simulink model "HybridControllerP2C2ahm"  (R2024b)
settings: Solver=FixedStepDiscrete  StartTime=0.0  StopTime=inf  FixedStep=controlPeriod  RelTol=1e-3
PreLoadFcn:
  | initializeSimulation;
InitFcn:
  | clear('all');
  | initializeSimulation;
values from neighbouring files (symbols this model uses):
  MRC = [2 0.05 0.001]./10    [ATS_setup.m]
  Nl = floor(tl/controlPeriod)    [ATS_setup.m]
  P_range = [0.9 1.1 ... (first row only)    [ATS_setup.m]
  Par = zeros(3,HybridCtrlParameters.nDOF)    [ATS_setup.m]
  SN = 16    [ATS_setup.m]
  Threshold = zeros(1,HybridCtrlParameters.nDOF)    [ATS_setup.m]
  Zden = zsys.Denominator{1}    [ATS_setup.m]
  Znum = zsys.Numerator{1}    [ATS_setup.m]
undefined symbols (not defined in the file or in its folder): HybridCtrlParameters
libraries: simulink x11
settings Model: Creator=mcdevin  LastModifiedBy=Andreas
settings SFSimCC: SimCustomHeaderCode="#include \"PredictorCorrector.h\""  SimUserSources=PredictorCorrector.c

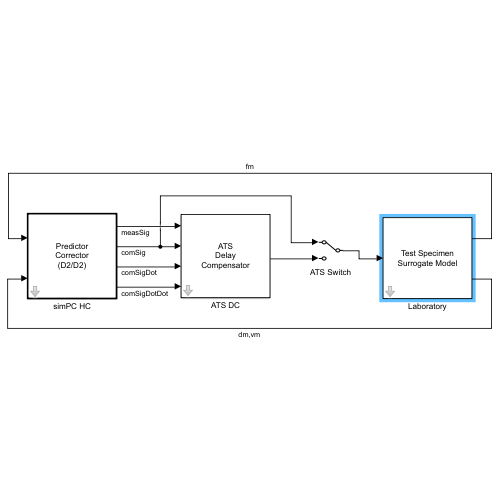
[thumbnail: Simulink's stored preview of the top-level diagram]
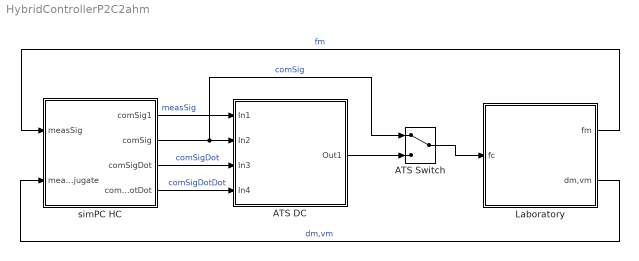
== system HybridControllerP2C2ahm ==
  ATS DC : Subsystem
      mask Display: disp('ATS\nDelay\nCompensator')
  ATS Switch : ManualSwitch
  Laboratory : Subsystem
      mask Display: disp('Test Specimen\nSurrogate Model')
  simPC HC : Subsystem  mask(Hybrid Controller: D2/D2){hcp=HybridCtrlParameters}
      mask prompts: hcp "Hybrid control parameter structure :"
      mask help: Hybrid Controller using C0-continuous quadratic Lagrange interpolation for prediction and correction
      mask init:
      | if isfield(hcp,'nDOF')
      |     nDOF = hcp.nDOF;
      | else
      |     nDOF = 1;
      | end
      | if isfield(hcp,'upFact')
      |     upFact = hcp.upFact;
      | else
      |     upFact = 1;
      | end
      | if isfield(hcp,'iDelay')
      |     iDelay = hcp.iDelay;
      | else
      |     iDelay = zeros(1,nDOF);
      | end
      | dtInt = hcp.dtInt;
      | dtSim = hcp.dtSim;
      | dtCon = hcp.dtCon;
      | N = hcp.N;
      mask Display: disp('Predictor\nCorrector\n(D2/D2)')
  wires:
  ATS DC/1(Out1) -> ATS Switch/2
  simPC HC/1(comSig1) -> ATS DC/1(In1)  "measSig"
  simPC HC/4(comSigDotDot) -> ATS DC/4(In4)  "comSigDotDot"
  simPC HC/2(comSig) -> ATS Switch/1, ATS DC/2(In2)  "comSig"
  simPC HC/3(comSigDot) -> ATS DC/3(In3)  "comSigDot"
  ATS Switch/1 -> Laboratory/1(fc)
  Laboratory/2(dm,vm) -> simPC HC/2(measSigConjugate)  "dm,vm"
  Laboratory/1(fm) -> simPC HC/1(measSig)  "fm"

== system HybridControllerP2C2ahm/ATS DC ==
  In1 : Inport
  In2 : Inport  Port=2
  In3 : Inport  Port=3
  In4 : Inport  Port=4
  ATS Compensator : Subsystem  mask(Adaptive Time Series (ATS) Compensator){param=Par, threshold=Threshold}
      mask prompts: param "Initial a0, a1, a2 values :"; threshold "Threshold for triggering :"
      mask help:
      | by Yunbyeong Chae, Old Dominion University
      | Ref: Chae, Y., Kazemibidokhti, K., and Ricles, J.M. (2013)
      | “Adaptive time series compensator for delay compensation of servo-hydraulic actuator systems for real-time hybrid simulation”,
      | Earthquake Engineering and Structural Dynamics, 42(11), 1697-1715.
  Subsystem : Subsystem
      mask Display: disp('Recorder')
  Out1 : Outport  VectorParamsAs1DForOutWhenUnconnected=off
  wires:
  ATS Compensator/2(apar) -> Subsystem/2(In2)
  ATS Compensator/1(compSig) -> Out1/1, Subsystem/1(In1)
  In1/1 -> ATS Compensator/1(measSig)
  In2/1 -> ATS Compensator/2(comSig)
  In3/1 -> ATS Compensator/3(comSigDot)
  In4/1 -> ATS Compensator/4(comSigDotDot)

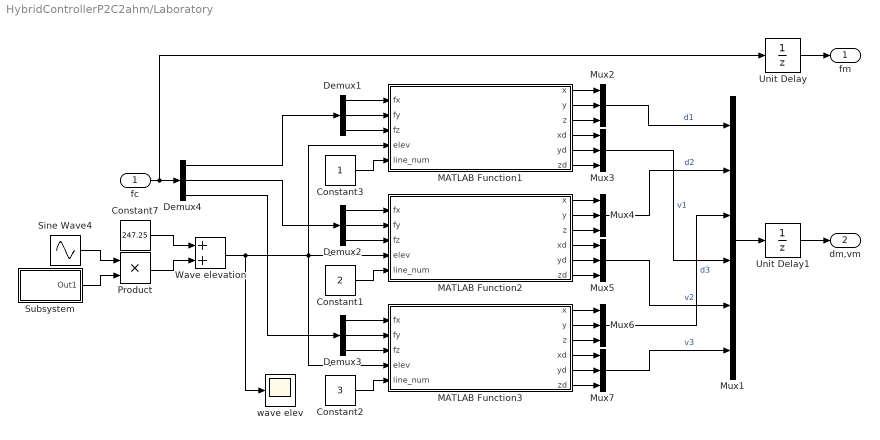
== system HybridControllerP2C2ahm/Laboratory ==
  fc : Inport
  Constant1 : Constant  Value=2
  Constant2 : Constant  Value=3
  Constant3 : Constant
  Constant7 : Constant  Value=247.25
  Demux{1..4} (4 alike) : Demux  Outputs=3
  MATLAB Function1 : MATLAB Function  TreatAsAtomicUnit=on
  MATLAB Function2 : MATLAB Function  TreatAsAtomicUnit=on
  MATLAB Function3 : MATLAB Function  TreatAsAtomicUnit=on
  Mux1 : Mux  Inputs=6
  Mux{2..7} (6 alike) : Mux  Inputs=3
  Product : Product
  Sine Wave4 : Sin  Amplitude=0.5  Frequency=2*pi/6  SampleTime=0
  Subsystem : Subsystem  mask{startTime=0.5, rampTime=1, initOut=0}
      mask prompts: startTime "Start time:"; rampTime "Ramp time:"; initOut "Initial output:"
      mask DialogControl DescTextVar Prompt: Output a Cosine bell ramp signal starting at the specified time.
      mask Display: fprintf('Cosine Bell\nRamp')
  Unit Delay : UnitDelay  SampleTime=-1  HasFrameUpgradeWarning=on
  Unit Delay1 : UnitDelay  SampleTime=-1  HasFrameUpgradeWarning=on
  Wave elevation : Sum
  wave elev : Scope
  fm : Outport
  dm,vm : Outport  Port=2
  wires:
  Constant7/1 -> Wave elevation/1
  Demux2/3 -> MATLAB Function2/3(fz)
  MATLAB Function2/6(zd) -> Mux5/3
  Demux1/3 -> MATLAB Function1/3(fz)
  Wave elevation/1 -> wave elev/1, MATLAB Function1/4(elev), MATLAB Function2/4(elev), MATLAB Function3/4(elev)
  Demux4/1 -> Demux1/1
  Demux2/2 -> MATLAB Function2/2(fy)
  Demux2/1 -> MATLAB Function2/1(fx)
  MATLAB Function1/5(yd) -> Mux3/2
  MATLAB Function2/3(z) -> Mux4/3
  Mux4/1 -> Mux1/2  "d2"
  Constant1/1 -> MATLAB Function2/5(line_num)
  Demux3/1 -> MATLAB Function3/1(fx)
  MATLAB Function3/1(x) -> Mux6/1
  MATLAB Function1/1(x) -> Mux2/1
  Mux7/1 -> Mux1/6  "v3"
  Constant2/1 -> MATLAB Function3/5(line_num)
  MATLAB Function3/4(xd) -> Mux7/1
  Demux3/3 -> MATLAB Function3/3(fz)
  Mux5/1 -> Mux1/5  "v2"
  Demux3/2 -> MATLAB Function3/2(fy)
  Mux3/1 -> Mux1/4  "v1"
  MATLAB Function2/2(y) -> Mux4/2
  MATLAB Function1/2(y) -> Mux2/2
  Demux1/1 -> MATLAB Function1/1(fx)
  MATLAB Function1/3(z) -> Mux2/3
  MATLAB Function3/2(y) -> Mux6/2
  MATLAB Function1/6(zd) -> Mux3/3
  Mux2/1 -> Mux1/1  "d1"
  MATLAB Function3/3(z) -> Mux6/3
  Demux1/2 -> MATLAB Function1/2(fy)
  MATLAB Function2/5(yd) -> Mux5/2
  Constant3/1 -> MATLAB Function1/5(line_num)
  MATLAB Function2/4(xd) -> Mux5/1
  MATLAB Function3/6(zd) -> Mux7/3
  Demux4/3 -> Demux3/1
  MATLAB Function2/1(x) -> Mux4/1
  MATLAB Function3/5(yd) -> Mux7/2
  Mux6/1 -> Mux1/3  "d3"
  MATLAB Function1/4(xd) -> Mux3/1
  Demux4/2 -> Demux2/1
  fc/1 -> Unit Delay/1, Demux4/1
  Mux1/1 -> Unit Delay1/1
  Unit Delay/1 -> fm/1
  Unit Delay1/1 -> dm,vm/1
  Sine Wave4/1 -> Product/1
  Subsystem/1(Out1) -> Product/2
  Product/1 -> Wave elevation/2

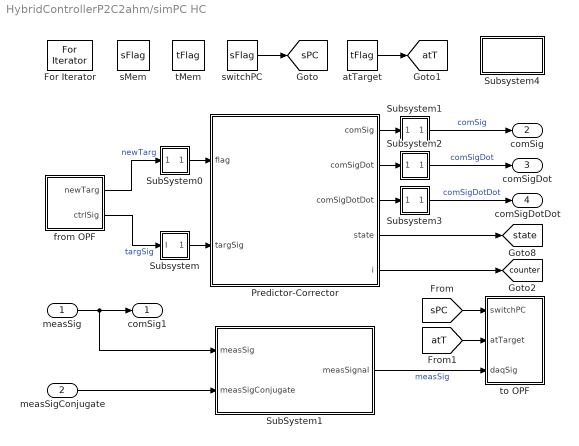
== system HybridControllerP2C2ahm/simPC HC ==
  measSig : Inport
  measSigConjugate : Inport  Port=2
  For Iterator : ForIterator  IterationLimit=upFact  ShowIterationPort=off
  Predictor-Corrector : Stateflow chart  TreatAsAtomicUnit=on
  SubSystem0 : Subsystem
      mask Display: disp('I/O')
  SubSystem1 : Subsystem
  Subsystem : Subsystem
      mask Display: disp('I/O')
  Subsystem1 : Subsystem
      mask Display: disp('I/O')
  Subsystem2 : Subsystem
      mask Display: disp('I/O')
  Subsystem3 : Subsystem
      mask Display: disp('I/O')
  Subsystem4 : Subsystem
      mask Display: disp('Recorder')
  atTarget : DataStoreRead  DataStoreName=tFlag  IndexOptions=Index vector (dialog)  Indices=1  OutputSizes=1
  from OPF : Subsystem
  sMem : DataStoreMemory  DataStoreName=sFlag  ShowAdditionalParam=off  OutDataTypeStr=int32
  switchPC : DataStoreRead  DataStoreName=sFlag  IndexOptions=Index vector (dialog)  Indices=1  OutputSizes=1
  tMem : DataStoreMemory  DataStoreName=tFlag  ShowAdditionalParam=off  OutDataTypeStr=int32
  to OPF : Subsystem
  comSig1 : Outport  VectorParamsAs1DForOutWhenUnconnected=off
  comSig : Outport  Port=2  VectorParamsAs1DForOutWhenUnconnected=off
  comSigDot : Outport  Port=3  VectorParamsAs1DForOutWhenUnconnected=off
  comSigDotDot : Outport  Port=4  VectorParamsAs1DForOutWhenUnconnected=off
  tag scope: atT=global, counter=global, sPC=global, state=global
  wires:
  SubSystem1/1(measSignal) -> to OPF/3(daqSig)  "measSig"
  Predictor-Corrector/5(i) -> [counter]
  SubSystem0/1(Out) -> Predictor-Corrector/1(flag)
  from OPF/1(newTarg) -> SubSystem0/1(In)  "newTarg"
  switchPC/1 -> [sPC]
  atTarget/1 -> [atT]
  Subsystem/1(O) -> Predictor-Corrector/2(targSig)
  measSig/1 -> SubSystem1/1(measSig), comSig1/1
  measSigConjugate/1 -> SubSystem1/2(measSigConjugate)
  Predictor-Corrector/1(comSig) -> Subsystem1/1(In)
  Predictor-Corrector/2(comSigDot) -> Subsystem2/1(In)
  Predictor-Corrector/3(comSigDotDot) -> Subsystem3/1(In)
  from OPF/2(ctrlSig) -> Subsystem/1(I)  "targSig"
  Predictor-Corrector/4(state) -> [state]
  Subsystem2/1(Out) -> comSigDot/1  "comSigDot"
  Subsystem3/1(Out) -> comSigDotDot/1  "comSigDotDot"
  Subsystem1/1(Out) -> comSig/1  "comSig"
  [sPC] -> to OPF/1(switchPC)
  [atT] -> to OPF/2(atTarget)

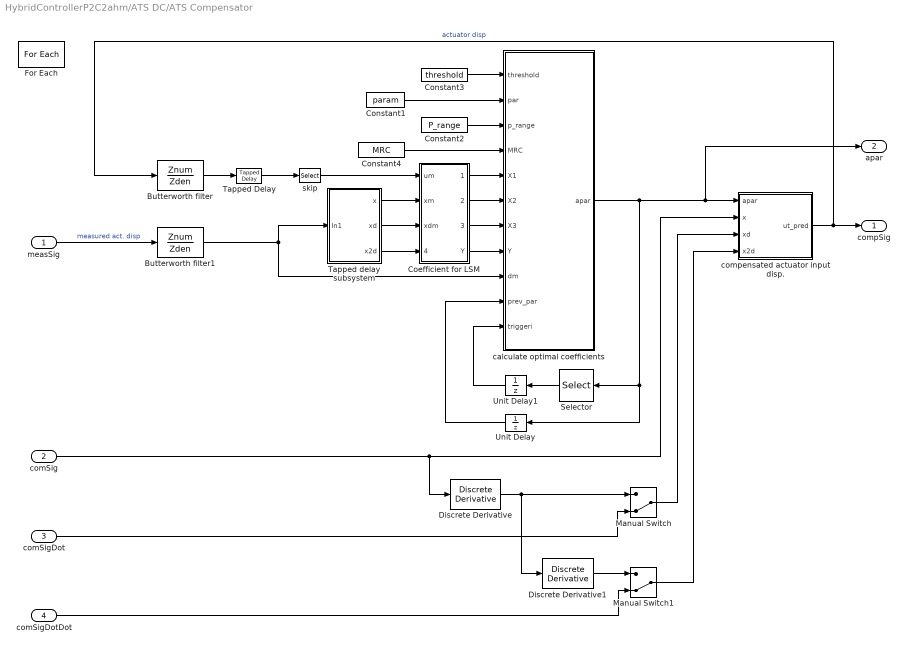
== system HybridControllerP2C2ahm/ATS DC/ATS Compensator ==
  measSig : Inport  Partition=on  PartitionDimension=1  PartitionWidth=1  PartitionOffset=0
  comSig : Inport  Port=2  Partition=on  PartitionDimension=1  PartitionWidth=1  PartitionOffset=0
  comSigDot : Inport  Port=3  Partition=on  PartitionDimension=1  PartitionWidth=1  PartitionOffset=0
  comSigDotDot : Inport  Port=4  Partition=on  PartitionDimension=1  PartitionWidth=1  PartitionOffset=0
  Butterworth filter : DiscreteTransferFcn  Numerator=Znum  Denominator=Zden
  Butterworth filter1 : DiscreteTransferFcn  Numerator=Znum  Denominator=Zden
  Coefficient for LSM : Subsystem
  Constant1 : Constant  Value=param
  Constant2 : Constant  Value=P_range
  Constant3 : Constant  Value=threshold
  Constant4 : Constant  Value=MRC
  Discrete Derivative : simulink/Discrete/Discrete Derivative  gainval=1.0  ICPrevScaledInput=0.0  OutMin=[]  OutMax=[]  OutDataType=fixdt(1, 16)  OutScaling=2^-10  DoSatur=off
  Discrete Derivative1 : simulink/Discrete/Discrete Derivative  gainval=1.0  ICPrevScaledInput=0.0  OutMin=[]  OutMax=[]  OutDataType=fixdt(1, 16)  OutScaling=2^-10  DoSatur=off
  For Each : ForEach  DisableCoverage=on  IterateSubsysMaskParameter=on,on  SubsysMaskParameterIterationDimension=2,2
  Manual Switch : ManualSwitch  CurrentSetting=0
  Manual Switch1 : ManualSwitch  CurrentSetting=0
  Selector : Selector  InputPortWidth=4  IndexOptions=Index vector (dialog)  Indices=4  OutputSizes=1
  Tapped Delay : simulink/Discrete/Tapped Delay  vinit=0.0  samptime=-1  NumDelays=Nl  DelayOrder=Oldest  includeCurrent=off
  Tapped delay subsystem : Subsystem
  Unit Delay : UnitDelay  SampleTime=-1  HasFrameUpgradeWarning=on
  Unit Delay1 : UnitDelay  SampleTime=-1  HasFrameUpgradeWarning=on
  calculate optimal coefficients : MATLAB Function  TreatAsAtomicUnit=on
  compensated actuator input disp. : MATLAB Function  TreatAsAtomicUnit=on
  skip : Selector  InputPortWidth=Nl  IndexOptions=Index vector (dialog)  Indices=[1:SN:Nl]  OutputSizes=1
  compSig : Outport  ConcatenationDimension=1  VectorParamsAs1DForOutWhenUnconnected=off
  apar : Outport  Port=2  ConcatenationDimension=1  VectorParamsAs1DForOutWhenUnconnected=off
  wires:
  measSig/1 -> Butterworth filter1/1  "measured act. disp"
  Tapped Delay/1 -> skip/1
  calculate optimal coefficients/1(apar) -> Unit Delay/1, Selector/1, apar/1, compensated actuator input disp./1(apar)
  compensated actuator input disp./1(ut_pred) -> compSig/1, Butterworth filter/1  "actuator disp"
  Constant1/1 -> calculate optimal coefficients/2(par)
  Constant2/1 -> calculate optimal coefficients/3(p_range)
  Unit Delay/1 -> calculate optimal coefficients/10(prev_par)
  comSig/1 -> compensated actuator input disp./2(x), Discrete Derivative/1
  skip/1 -> Coefficient for LSM/1(um)
  Tapped delay subsystem/1(x) -> Coefficient for LSM/2(xm)
  Tapped delay subsystem/2(xd) -> Coefficient for LSM/3(xdm)
  Tapped delay subsystem/3(x2d) -> Coefficient for LSM/4(x2dm)
  Coefficient for LSM/1(X(1,:)) -> calculate optimal coefficients/5(X1)
  Coefficient for LSM/2(X(2,:)) -> calculate optimal coefficients/6(X2)
  Coefficient for LSM/3(X(3,:)) -> calculate optimal coefficients/7(X3)
  Coefficient for LSM/4(Y) -> calculate optimal coefficients/8(Y)
  Unit Delay1/1 -> calculate optimal coefficients/11(triggeri)
  Constant3/1 -> calculate optimal coefficients/1(threshold)
  Butterworth filter/1 -> Tapped Delay/1
  Constant4/1 -> calculate optimal coefficients/4(MRC)
  Selector/1 -> Unit Delay1/1
  Manual Switch/1 -> compensated actuator input disp./3(xd)
  Discrete Derivative/1 -> Manual Switch/1, Discrete Derivative1/1
  comSigDot/1 -> Manual Switch/2
  Discrete Derivative1/1 -> Manual Switch1/1
  Manual Switch1/1 -> compensated actuator input disp./4(x2d)
  comSigDotDot/1 -> Manual Switch1/2
  Butterworth filter1/1 -> Tapped delay subsystem/1(In1), calculate optimal coefficients/9(dm)

== system HybridControllerP2C2ahm/ATS DC/Subsystem ==
  In1 : Inport
  In2 : Inport  Port=2
  Mux : Mux  Inputs=2
  wires:
  In1/1 -> Mux/1
  Mux/1 -> ?
  In2/1 -> Mux/2

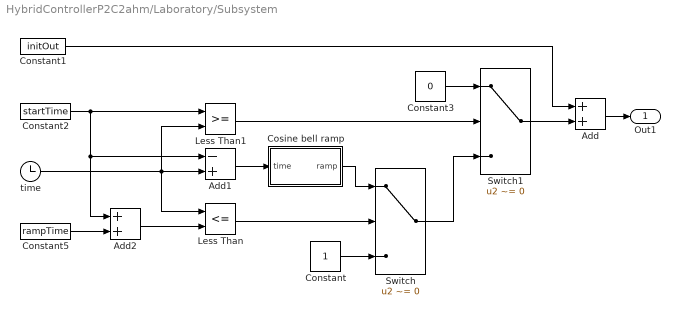
== system HybridControllerP2C2ahm/Laboratory/Subsystem ==
  Add : Sum
  Add1 : Sum  Inputs=-+
  Add2 : Sum
  Constant : Constant
  Constant1 : Constant  Value=initOut
  Constant2 : Constant  Value=startTime
  Constant3 : Constant  Value=0
  Constant5 : Constant  Value=rampTime
  Cosine bell ramp : Subsystem
  Less Than : RelationalOperator  Operator=<=  OutDataTypeStr=boolean  RndMeth=Simplest  InputSameDT=off
  Less Than1 : RelationalOperator  OutDataTypeStr=boolean  RndMeth=Simplest  InputSameDT=off
  Switch : Switch  Criteria=u2 ~= 0  SaturateOnIntegerOverflow=off  InputSameDT=off
  Switch1 : Switch  Criteria=u2 ~= 0  SaturateOnIntegerOverflow=off  InputSameDT=off
  time : Clock
  Out1 : Outport
  wires:
  Less Than1/1 -> Switch1/2
  Constant3/1 -> Switch1/1
  Switch/1 -> Switch1/3
  time/1 -> Less Than1/2, Less Than/1, Add1/2
  Constant2/1 -> Add1/1, Add2/1, Less Than1/1
  Constant1/1 -> Add/1
  Switch1/1 -> Add/2
  Add/1 -> Out1/1
  Cosine bell ramp/1(ramp) -> Switch/1
  Constant/1 -> Switch/3
  Less Than/1 -> Switch/2
  Add1/1 -> Cosine bell ramp/1(time)
  Add2/1 -> Less Than/2
  Constant5/1 -> Add2/2

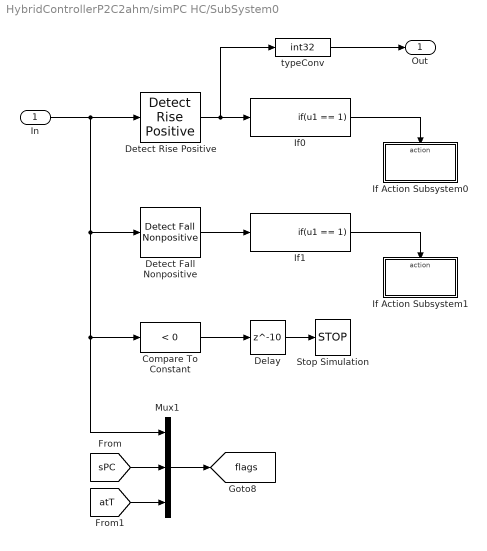
== system HybridControllerP2C2ahm/simPC HC/SubSystem0 ==
  In : Inport
  Compare To Constant : simulink/Logic and Bit Operations/Compare To Constant  relop=<  const=0  OutDataTypeStr=boolean
  Delay : Delay  DelayLength=10
  Detect Fall Nonpositive : simulink/Logic and Bit Operations/Detect Fall Nonpositive  vinit=0  OutDataTypeStr=uint8
  Detect Rise Positive : simulink/Logic and Bit Operations/Detect Rise Positive  vinit=0  OutDataTypeStr=uint8
  If Action Subsystem0 : Subsystem  TreatAsAtomicUnit=on
  If Action Subsystem1 : Subsystem  TreatAsAtomicUnit=on
  If0 : If  IfExpression=u1 == 1  ShowElse=off
  If1 : If  IfExpression=u1 == 1  ShowElse=off
  Mux1 : Mux  Inputs=3
  Stop Simulation : Stop
  typeConv : DataTypeConversion  OutDataTypeStr=int32
  Out : Outport  VectorParamsAs1DForOutWhenUnconnected=off
  tag scope: flags=global
  wires:
  Detect Rise Positive/1 -> If0/1, typeConv/1
  Detect Fall Nonpositive/1 -> If1/1
  If1/1 -> If Action Subsystem1/Action
  If0/1 -> If Action Subsystem0/Action
  typeConv/1 -> Out/1
  Mux1/1 -> [flags]
  [sPC] -> Mux1/2
  [atT] -> Mux1/3
  In/1 -> Detect Rise Positive/1, Detect Fall Nonpositive/1, Compare To Constant/1, Mux1/1
  Compare To Constant/1 -> Delay/1
  Delay/1 -> Stop Simulation/1

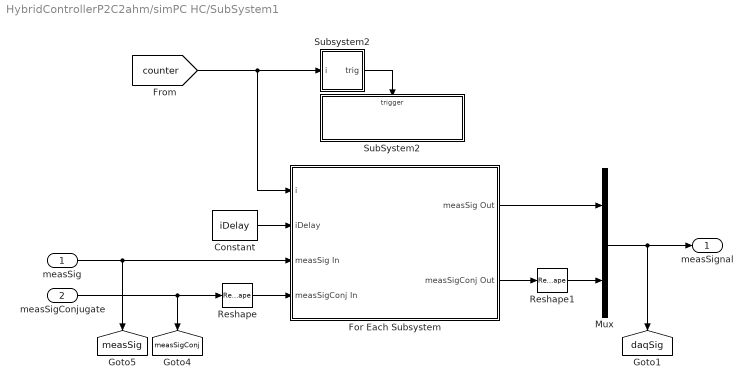
== system HybridControllerP2C2ahm/simPC HC/SubSystem1 ==
  measSig : Inport
  measSigConjugate : Inport  Port=2
  Constant : Constant  Value=iDelay
  For Each Subsystem : Subsystem  TreatAsAtomicUnit=on
  Mux : Mux  Inputs=2
  Reshape : Reshape  OutputDimensionality=Customize  OutputDimensions=[nDOF,2]
  Reshape1 : Reshape  OutputDimensions=[nDOF,2]
  SubSystem2 : Subsystem  TreatAsAtomicUnit=on
  Subsystem2 : Subsystem
  measSignal : Outport  VectorParamsAs1DForOutWhenUnconnected=off
  tag scope: daqSig=global, measSig=global, measSigConj=global
  wires:
  Subsystem2/1(trig) -> SubSystem2/Trigger
  [counter] -> Subsystem2/1(i), For Each Subsystem/1(i)
  Constant/1 -> For Each Subsystem/2(iDelay)
  measSig/1 -> For Each Subsystem/3(measSig In), [measSig]
  measSigConjugate/1 -> Reshape/1, [measSigConj]
  For Each Subsystem/1(measSig Out) -> Mux/1
  For Each Subsystem/2(measSigConj Out) -> Reshape1/1
  Mux/1 -> measSignal/1, [daqSig]
  Reshape/1 -> For Each Subsystem/4(measSigConj In)
  Reshape1/1 -> Mux/2

== system HybridControllerP2C2ahm/simPC HC/Subsystem ==
  I : Inport  PortDimensions=nDOF
  Dummy Aug : Mux  Inputs=[nDOF 1]
  Dummy Zero : Constant  Value=0  OutDataTypeStr=double  SampleTime=-1
  O : Outport  PortDimensions=nDOF+1  VectorParamsAs1DForOutWhenUnconnected=off
  tag scope: targSig=global
  wires:
  Dummy Zero/1 -> Dummy Aug/2
  I/1 -> Dummy Aug/1, [targSig]
  Dummy Aug/1 -> O/1

== system HybridControllerP2C2ahm/simPC HC/Subsystem1 ==
  In : Inport  PortDimensions=nDOF+1
  Dummy Trn : Demux  Outputs=[nDOF 1]
  Terminator3 : Terminator
  Out : Outport  PortDimensions=nDOF  VectorParamsAs1DForOutWhenUnconnected=off
  tag scope: comSig=global
  wires:
  Dummy Trn/2 -> Terminator3/1
  Dummy Trn/1 -> Out/1, [comSig]
  In/1 -> Dummy Trn/1

== system HybridControllerP2C2ahm/simPC HC/Subsystem2 ==
  In : Inport  PortDimensions=nDOF+1
  Dummy Trn : Demux  Outputs=[nDOF 1]
  Terminator3 : Terminator
  Out : Outport  PortDimensions=nDOF  VectorParamsAs1DForOutWhenUnconnected=off
  tag scope: comSigDot=global
  wires:
  Dummy Trn/2 -> Terminator3/1
  Dummy Trn/1 -> Out/1, [comSigDot]
  In/1 -> Dummy Trn/1

== system HybridControllerP2C2ahm/simPC HC/Subsystem3 ==
  In : Inport  PortDimensions=nDOF+1
  Dummy Trn : Demux  Outputs=[nDOF 1]
  Terminator3 : Terminator
  Out : Outport  PortDimensions=nDOF  VectorParamsAs1DForOutWhenUnconnected=off
  tag scope: comSigDotDot=global
  wires:
  Dummy Trn/2 -> Terminator3/1
  Dummy Trn/1 -> Out/1, [comSigDotDot]
  In/1 -> Dummy Trn/1

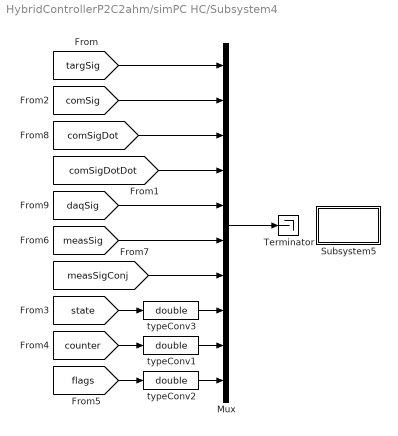
== system HybridControllerP2C2ahm/simPC HC/Subsystem4 ==
  Mux : Mux  Inputs=10
  Subsystem5 : Subsystem
      mask Display: disp('Scopes')
  Terminator : Terminator
  typeConv1 : DataTypeConversion  OutDataTypeStr=double
  typeConv2 : DataTypeConversion  OutDataTypeStr=double
  typeConv3 : DataTypeConversion  OutDataTypeStr=double
  wires:
  [flags] -> typeConv2/1
  [counter] -> typeConv1/1
  [state] -> typeConv3/1
  typeConv3/1 -> Mux/8
  typeConv1/1 -> Mux/9
  typeConv2/1 -> Mux/10
  [measSigConj] -> Mux/7
  [measSig] -> Mux/6
  [comSigDotDot] -> Mux/4
  [comSigDot] -> Mux/3
  [comSig] -> Mux/2
  [targSig] -> Mux/1
  Mux/1 -> Terminator/1
  [daqSig] -> Mux/5

== system HybridControllerP2C2ahm/simPC HC/from OPF ==
  S-Function1 : S-Function  FunctionName=SFun_OPF_TCPServer  Parameters=22222, numCtrlSignals, numDaqSignals, nbMode  SFunctionDeploymentMode=off  EnableBusSupport=off  mask(OpenFresco Connect: TCP Server){ipPort=22222, numCtrlSignals=nDOF, numDaqSignals=3*nDOF, nbMode=on}
      mask prompts: ipPort "IP Port Number of Server :"; numCtrlSignals "Number of Control Signals :"; numDaqSignals "Number of DAQ Signals :"; nbMode "Nonblocking mode"
      mask help: Server block to connect with the "SimSimulink" experimental control in OpenFresco using a TCP socket.
      mask Display: disp('OpenFresco\nConnect\nTCP Server');
  Unit Delay : UnitDelay  SampleTime=-1  HasFrameUpgradeWarning=on
  typeConv : DataTypeConversion  OutDataTypeStr=double  RndMeth=Round
  typeConv1 : DataTypeConversion  OutDataTypeStr=double  RndMeth=Round
  typeConv2 : DataTypeConversion  OutDataTypeStr=int32  RndMeth=Round
  newTarg : Outport  VectorParamsAs1DForOutWhenUnconnected=off
  ctrlSig : Outport  Port=2  PortDimensions=nDOF  VectorParamsAs1DForOutWhenUnconnected=off
  wires:
  typeConv2/1 -> newTarg/1
  S-Function1/1 -> typeConv2/1
  S-Function1/2 -> ctrlSig/1
  typeConv1/1 -> S-Function1/2
  typeConv/1 -> S-Function1/1
  [atT] -> typeConv1/1
  [sPC] -> typeConv/1
  [daqSig] -> Unit Delay/1
  Unit Delay/1 -> S-Function1/3

== system HybridControllerP2C2ahm/simPC HC/to OPF ==
  note: See "from OPF" block
  switchPC : Inport
  atTarget : Inport  Port=2
  daqSig : Inport  Port=3
  Terminator : Terminator
  Terminator1 : Terminator
  Terminator2 : Terminator
  wires:
  switchPC/1 -> Terminator/1
  atTarget/1 -> Terminator1/1
  daqSig/1 -> Terminator2/1

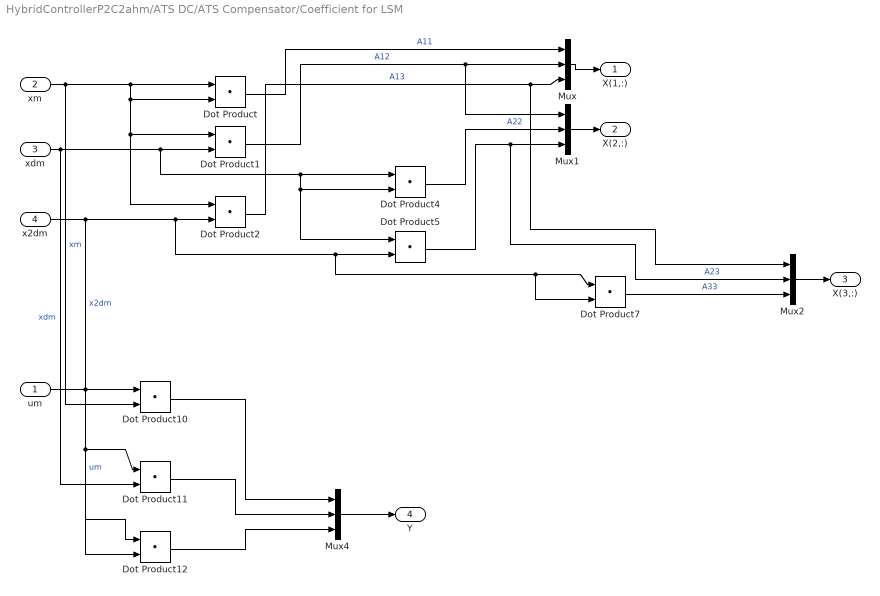
== system HybridControllerP2C2ahm/ATS DC/ATS Compensator/Coefficient for LSM ==
  um : Inport
  xm : Inport  Port=2
  xdm : Inport  Port=3
  x2dm : Inport  Port=4
  Dot Product{,1..2,4..5,7,10..12} (9 alike) : DotProduct  OutDataTypeStr=Inherit: Inherit via internal rule
  Mux{,1..2,4} (4 alike) : Mux  Inputs=3
  X(1,:) : Outport  VectorParamsAs1DForOutWhenUnconnected=off
  X(2,:) : Outport  Port=2  VectorParamsAs1DForOutWhenUnconnected=off
  X(3,:) : Outport  Port=3  VectorParamsAs1DForOutWhenUnconnected=off
  Y : Outport  Port=4  VectorParamsAs1DForOutWhenUnconnected=off
  wires:
  xm/1 -> Dot Product/1, Dot Product/2, Dot Product1/1, Dot Product2/1, Dot Product10/2  "xm"
  xdm/1 -> Dot Product1/2, Dot Product4/1, Dot Product4/2, Dot Product5/1, Dot Product11/2  "xdm"
  x2dm/1 -> Dot Product2/2, Dot Product5/2, Dot Product7/1, Dot Product7/2, Dot Product12/2  "x2dm"
  um/1 -> Dot Product10/1, Dot Product11/1, Dot Product12/1  "um"
  Dot Product/1 -> Mux/1  "A11"
  Dot Product1/1 -> Mux/2, Mux1/1  "A12"
  Dot Product2/1 -> Mux/3, Mux2/1  "A13"
  Mux/1 -> X(1,:)/1
  Dot Product4/1 -> Mux1/2  "A22"
  Dot Product5/1 -> Mux1/3, Mux2/2  "A23"
  Mux1/1 -> X(2,:)/1
  Dot Product7/1 -> Mux2/3  "A33"
  Mux2/1 -> X(3,:)/1
  Mux4/1 -> Y/1
  Dot Product10/1 -> Mux4/1
  Dot Product11/1 -> Mux4/2
  Dot Product12/1 -> Mux4/3

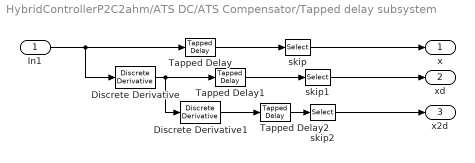
== system HybridControllerP2C2ahm/ATS DC/ATS Compensator/Tapped delay subsystem ==
  In1 : Inport
  Discrete Derivative : simulink/Discrete/Discrete Derivative  gainval=1.0  ICPrevScaledInput=0.0  OutMin=[]  OutMax=[]  OutDataType=fixdt(1, 16)  OutScaling=2^-10  DoSatur=off
  Discrete Derivative1 : simulink/Discrete/Discrete Derivative  gainval=1.0  ICPrevScaledInput=0.0  OutMin=[]  OutMax=[]  OutDataType=fixdt(1, 16)  OutScaling=2^-10  DoSatur=off
  Tapped Delay : simulink/Discrete/Tapped Delay  vinit=0.0  samptime=-1  NumDelays=Nl  DelayOrder=Oldest  includeCurrent=off
  Tapped Delay1 : simulink/Discrete/Tapped Delay  vinit=0.0  samptime=-1  NumDelays=Nl  DelayOrder=Oldest  includeCurrent=off
  Tapped Delay2 : simulink/Discrete/Tapped Delay  vinit=0.0  samptime=-1  NumDelays=Nl  DelayOrder=Oldest  includeCurrent=off
  skip : Selector  InputPortWidth=Nl  IndexOptions=Index vector (dialog)  Indices=[1:SN:Nl]  OutputSizes=1
  skip1 : Selector  InputPortWidth=Nl  IndexOptions=Index vector (dialog)  Indices=[1:SN:Nl]  OutputSizes=1
  skip2 : Selector  InputPortWidth=Nl  IndexOptions=Index vector (dialog)  Indices=[1:SN:Nl]  OutputSizes=1
  x : Outport  VectorParamsAs1DForOutWhenUnconnected=off
  xd : Outport  Port=2  VectorParamsAs1DForOutWhenUnconnected=off
  x2d : Outport  Port=3  VectorParamsAs1DForOutWhenUnconnected=off
  wires:
  In1/1 -> Discrete Derivative/1, Tapped Delay/1
  Discrete Derivative/1 -> Discrete Derivative1/1, Tapped Delay1/1
  Discrete Derivative1/1 -> Tapped Delay2/1
  Tapped Delay/1 -> skip/1
  Tapped Delay1/1 -> skip1/1
  Tapped Delay2/1 -> skip2/1
  skip/1 -> x/1
  skip1/1 -> xd/1
  skip2/1 -> x2d/1

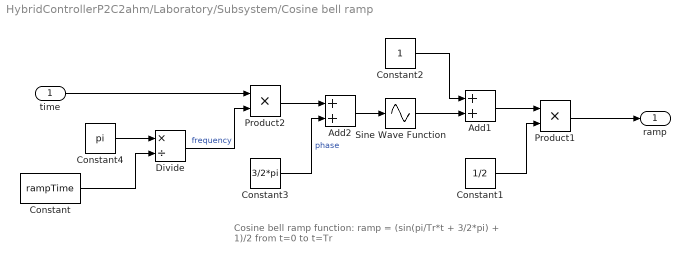
== system HybridControllerP2C2ahm/Laboratory/Subsystem/Cosine bell ramp ==
  note: Cosine bell ramp function:
      | ramp = (sin(pi/Tr*t + 3/2*pi) + 1)/2    from t=0 to t=Tr
  time : Inport
  Add1 : Sum
  Add2 : Sum
  Constant : Constant  Value=rampTime
  Constant1 : Constant  Value=1/2
  Constant2 : Constant
  Constant3 : Constant  Value=3/2*pi
  Constant4 : Constant  Value=pi
  Divide : Product  Inputs=*/
  Product1 : Product
  Product2 : Product
  Sine Wave Function : Sin  TimeSource=Use external signal  SampleTime=0
  ramp : Outport
  wires:
  Product1/1 -> ramp/1
  Constant2/1 -> Add1/1
  Constant3/1 -> Add2/2  "phase"
  Constant/1 -> Divide/2
  Divide/1 -> Product2/2  "frequency"
  Add1/1 -> Product1/1
  Constant4/1 -> Divide/1
  Add2/1 -> Sine Wave Function/1
  Product2/1 -> Add2/1
  time/1 -> Product2/1
  Sine Wave Function/1 -> Add1/2
  Constant1/1 -> Product1/2

== system HybridControllerP2C2ahm/simPC HC/SubSystem0/If Action Subsystem0 ==
  Action Port : ActionPort  PropagateVarSize=During execution  ActionPortLabel=if(u1 == 1)
  Data Store Write0 : DataStoreWrite  DataStoreName=sFlag  IndexOptions=Index vector (dialog)  Indices=1  OutputSizes=1
  Data Store Write1 : DataStoreWrite  DataStoreName=tFlag  IndexOptions=Index vector (dialog)  Indices=1  OutputSizes=1
  atTargetFlag : Constant  Value=0  OutDataTypeStr=int32  SampleTime=-1
  switchFlag : Constant  OutDataTypeStr=int32  SampleTime=-1
  wires:
  atTargetFlag/1 -> Data Store Write1/1
  switchFlag/1 -> Data Store Write0/1

== system HybridControllerP2C2ahm/simPC HC/SubSystem0/If Action Subsystem1 ==
  Action Port : ActionPort  PropagateVarSize=During execution  ActionPortLabel=if(u1 == 1)
  Data Store Write0 : DataStoreWrite  DataStoreName=sFlag  IndexOptions=Index vector (dialog)  Indices=1  OutputSizes=1
  switchFlag : Constant  Value=0  OutDataTypeStr=int32  SampleTime=-1
  wires:
  switchFlag/1 -> Data Store Write0/1

== system HybridControllerP2C2ahm/simPC HC/SubSystem1/For Each Subsystem ==
  i : Inport
  iDelay : Inport  Port=2  Partition=on  PartitionDimension=1  PartitionWidth=1  PartitionOffset=0
  measSig In : Inport  Port=3  Partition=on  PartitionDimension=1  PartitionWidth=1  PartitionOffset=0
  measSigConj In : Inport  Port=4  Partition=on  PartitionDimension=1  PartitionWidth=1  PartitionOffset=0
  For Each : ForEach  DisableCoverage=on
  SubSystem : Subsystem  TreatAsAtomicUnit=on
  Subsystem : Subsystem
  measSig Out : Outport  ConcatenationDimension=1  VectorParamsAs1DForOutWhenUnconnected=off
  measSigConj Out : Outport  Port=2  ConcatenationDimension=1  VectorParamsAs1DForOutWhenUnconnected=off
  wires:
  Subsystem/1(trig) -> SubSystem/Trigger
  measSig In/1 -> SubSystem/1(measSig In)
  measSigConj In/1 -> SubSystem/2(measSigC In)
  SubSystem/1(measSig Out) -> measSig Out/1
  SubSystem/2(measSigC Out) -> measSigConj Out/1
  iDelay/1 -> Subsystem/2(iDelay)
  i/1 -> Subsystem/1(i)

== system HybridControllerP2C2ahm/simPC HC/SubSystem1/SubSystem2 ==
  Trigger : TriggerPort  VariantControl=(inherit)
  Data Store Write : DataStoreWrite  DataStoreName=tFlag  IndexOptions=Index vector (dialog)  Indices=1  OutputSizes=1
  atTargetFlag : Constant  OutDataTypeStr=int32  SampleTime=-1
  wires:
  atTargetFlag/1 -> Data Store Write/1

== system HybridControllerP2C2ahm/simPC HC/SubSystem1/Subsystem2 ==
  i : Inport
  Add : Sum
  Constant : Constant  Value=max(iDelay)
  Constant1 : Constant  Value=N
  If : If  IfExpression=u1 == 0
  If Action Subsystem1 : Subsystem  TreatAsAtomicUnit=on
  If Action Subsystem2 : Subsystem  TreatAsAtomicUnit=on
  trig : Outport  VectorParamsAs1DForOutWhenUnconnected=off
  wires:
  Constant/1 -> If/1, If Action Subsystem2/2(In2)
  If/1 -> If Action Subsystem1/Action
  If/2 -> If Action Subsystem2/Action
  If Action Subsystem1/1(Out1) -> Add/1
  If Action Subsystem2/1(Out1) -> Add/2
  Add/1 -> trig/1
  i/1 -> If Action Subsystem1/2(In2), If Action Subsystem2/1(In1)
  Constant1/1 -> If Action Subsystem1/1(In1)

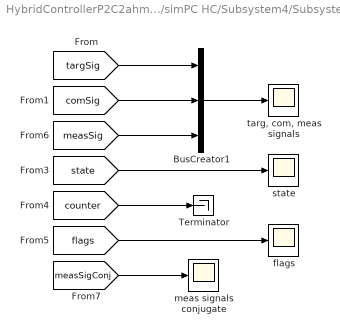
== system HybridControllerP2C2ahm/simPC HC/Subsystem4/Subsystem5 ==
  BusCreator1 : BusCreator  Inputs=3
  Terminator : Terminator
  flags : Scope
  meas signals conjugate : Scope
  state : Scope
  "targ, com, meas signals" : Scope
  wires:
  [targSig] -> BusCreator1/1
  [comSig] -> BusCreator1/2
  [flags] -> flags/1
  [measSig] -> BusCreator1/3
  BusCreator1/1 -> "targ, com, meas signals"/1
  [state] -> state/1
  [counter] -> Terminator/1
  [measSigConj] -> meas signals conjugate/1

== system HybridControllerP2C2ahm/simPC HC/SubSystem1/For Each Subsystem/SubSystem ==
  measSig In : Inport
  measSigC In : Inport  Port=2
  Trigger : TriggerPort  VariantControl=(inherit)
  measSig Out : Outport  InitialOutput=[0]  VectorParamsAs1DForOutWhenUnconnected=off
  measSigC Out : Outport  Port=2  InitialOutput=[0]  VectorParamsAs1DForOutWhenUnconnected=off
  wires:
  measSigC In/1 -> measSigC Out/1
  measSig In/1 -> measSig Out/1

== system HybridControllerP2C2ahm/simPC HC/SubSystem1/For Each Subsystem/Subsystem ==
  i : Inport
  iDelay : Inport  Port=2
  Add : Sum
  Constant1 : Constant  Value=N
  If : If  IfExpression=u1 == 0
  If Action Subsystem1 : Subsystem  TreatAsAtomicUnit=on
  If Action Subsystem2 : Subsystem  TreatAsAtomicUnit=on
  trig : Outport  VectorParamsAs1DForOutWhenUnconnected=off
  wires:
  iDelay/1 -> If/1, If Action Subsystem2/2(In2)
  If/1 -> If Action Subsystem1/Action
  If/2 -> If Action Subsystem2/Action
  If Action Subsystem1/1(Out1) -> Add/1
  If Action Subsystem2/1(Out1) -> Add/2
  Add/1 -> trig/1
  i/1 -> If Action Subsystem1/2(In2), If Action Subsystem2/1(In1)
  Constant1/1 -> If Action Subsystem1/1(In1)

== system HybridControllerP2C2ahm/simPC HC/SubSystem1/Subsystem2/If Action Subsystem1 ==
  In1 : Inport
  In2 : Inport  Port=2
  Action Port : ActionPort  ActionPortLabel=if(u1 == 0)
  Relational Operator : RelationalOperator  Operator===  OutDataTypeStr=boolean  InputSameDT=off
  Out1 : Outport  InitialOutput=0  VectorParamsAs1DForOutWhenUnconnected=off
  wires:
  Relational Operator/1 -> Out1/1
  In1/1 -> Relational Operator/1
  In2/1 -> Relational Operator/2

== system HybridControllerP2C2ahm/simPC HC/SubSystem1/Subsystem2/If Action Subsystem2 ==
  In1 : Inport
  In2 : Inport  Port=2
  Action Port : ActionPort  ActionPortLabel=else
  Relational Operator : RelationalOperator  Operator===  OutDataTypeStr=boolean  InputSameDT=off
  Out1 : Outport  InitialOutput=0  VectorParamsAs1DForOutWhenUnconnected=off
  wires:
  Relational Operator/1 -> Out1/1
  In1/1 -> Relational Operator/1
  In2/1 -> Relational Operator/2

== system HybridControllerP2C2ahm/simPC HC/SubSystem1/For Each Subsystem/Subsystem/If Action Subsystem1 ==
  In1 : Inport
  In2 : Inport  Port=2
  Action Port : ActionPort  ActionPortLabel=if(u1 == 0)
  Relational Operator : RelationalOperator  Operator===  OutDataTypeStr=boolean  InputSameDT=off
  Out1 : Outport  InitialOutput=0  VectorParamsAs1DForOutWhenUnconnected=off
  wires:
  Relational Operator/1 -> Out1/1
  In1/1 -> Relational Operator/1
  In2/1 -> Relational Operator/2

== system HybridControllerP2C2ahm/simPC HC/SubSystem1/For Each Subsystem/Subsystem/If Action Subsystem2 ==
  In1 : Inport
  In2 : Inport  Port=2
  Action Port : ActionPort  ActionPortLabel=else
  Relational Operator : RelationalOperator  Operator===  OutDataTypeStr=boolean  InputSameDT=off
  Out1 : Outport  InitialOutput=0  VectorParamsAs1DForOutWhenUnconnected=off
  wires:
  Relational Operator/1 -> Out1/1
  In1/1 -> Relational Operator/1
  In2/1 -> Relational Operator/2

== matlab function HybridControllerP2C2ahm/ATS DC/ATS Compensator/calculate optimal coefficients ==
  data: threshold input; par input; p_range input; MRC input; X1 input; apar output; X2 input; X3 input; Y input; dm input; prev_par input; triggeri input
function apar = fcn(threshold,par,p_range,MRC,X1,X2,X3,Y,dm,prev_par,triggeri)
%#codegen
%triggero=triggeri;
apar = [par; triggeri];

if( abs( dm ) > threshold || apar(4) )
    apar(4)=1;
    
    X = [X1 X2 X3];       
    
    temp=X\Y; 
    
    apar(1:3)=temp;
    
    if( isnan( apar(1) ) + isnan( apar(2) ) + isnan( apar(3) ) )
        apar=[par; triggeri];
    end
    
    
    % maximum change of rate
    if( abs(apar(1)-prev_par(1)) > MRC(1) )
        apar(1) = prev_par(1) + sign(apar(1)-prev_par(1))*MRC(1);
    end
    if( abs(apar(2)-prev_par(2)) > MRC(2) )
        apar(2) = prev_par(2) + sign(apar(2)-prev_par(2))*MRC(2);
    end
    if( abs(apar(3)-prev_par(3)) > MRC(3) )
        apar(3) = prev_par(3) + sign(apar(3)-prev_par(3))*MRC(3);
    end
    
    % limit of coefficients
    if( apar(1) < p_range(1,1) )
        apar(1) = p_range(1,1);
    end
    
    if( apar(1) > p_range(1,2) )
        apar(1) = p_range(1,2);
    end
    
    if( apar(2) < p_range(2,1) )
        apar(2) = p_range(2,1);
    end
    
    if( apar(2) > p_range(2,2) )
        apar(2) = p_range(2,2);
    end
    
    if( apar(3) < p_range(3,1) )
        apar(3) = p_range(3,1);
    end
    
    if( apar(3) > p_range(3,2) )
        apar(3) = p_range(3,2);
    end    
    
end

== matlab function HybridControllerP2C2ahm/ATS DC/ATS Compensator/compensated actuator input disp. ==
  data: apar input; x input; xd input; x2d input; ut_pred output
function ut_pred = fcn(apar,x,xd,x2d)
%#codegen

ut_pred = apar(1)*x + apar(2)*xd + apar(3)*x2d;

== matlab function HybridControllerP2C2ahm/Laboratory/MATLAB Function1 ==
  data: fx input; x output; fy input; fz input; elev input; line_num input; y output; z output; xd output; yd output; zd output
function [x, y, z, xd, yd, zd]  = SurrogateModel(fx, fy, fz, elev, line_num)
    
    % preallocate outputs
    x = double(0);
    y = double(0);
    z = double(0);
    xd = double(0);
    yd = double(0);
    zd = double(0);

    % declare python functions and inputs
    coder.extrinsic('py.list')
    coder.extrinsic('py.predict_motions.predict_motions');
    inputs = py.list({fx, fy, fz, elev});

    % set surrogate model files
    switch(line_num)
        case 1
            model_x = 'models/model_l1px.h5';
            model_y = 'models/model_l1py.h5';
            model_z = 'models/model_l1pz.h5';
            model_xd = 'models/model_l1vx.h5';
            model_yd = 'models/model_l1vy.h5';
            model_zd = 'models/model_l1vz.h5';
        case 2
            model_x = 'models/model_l2px.h5';
            model_y = 'models/model_l2py.h5';
            model_z = 'models/model_l2pz.h5';
            model_xd = 'models/model_l2vx.h5';
            model_yd = 'models/model_l2vy.h5';
            model_zd = 'models/model_l2vz.h5';
        case 3
            model_x = 'models/model_l3px.h5';
            model_y = 'models/model_l3py.h5';
            model_z = 'models/model_l3pz.h5';
            model_xd = 'models/model_l3vx.h5';
            model_yd = 'models/model_l3vy.h5';
            model_zd = 'models/model_l3vz.h5';
        otherwise
            error('Invalid line number.');
    end
    
    % call surrogate model to predict positions and velocities
    x_py = py.predict_motions.predict_motions(model_x, inputs);
    y_py = py.predict_motions.predict_motions(model_y, inputs);
    z_py = py.predict_motions.predict_motions(model_z, inputs);
    xd_py = py.predict_motions.predict_motions(model_xd, inputs);
    yd_py = py.predict_motions.predict_motions(model_yd, inputs);
    zd_py = py.predict_motions.predict_motions(model_zd, inputs);

    % convert Python outputs to MATLAB data types
    x = double(x_py);
    y = double(y_py);
    z = double(z_py);
    xd = double(xd_py);
    yd = double(yd_py);
    zd = double(zd_py);
    
end

== matlab function HybridControllerP2C2ahm/Laboratory/MATLAB Function2 ==
  data: fx input; x output; fy input; fz input; elev input; line_num input; y output; z output; xd output; yd output; zd output
function [x, y, z, xd, yd, zd]  = SurrogateModel(fx, fy, fz, elev, line_num)
    
    % preallocate outputs
    x = double(0);
    y = double(0);
    z = double(0);
    xd = double(0);
    yd = double(0);
    zd = double(0);

    % declare python functions and inputs
    coder.extrinsic('py.list')
    coder.extrinsic('py.predict_motions.predict_motions');
    inputs = py.list({fx, fy, fz, elev});

    % set surrogate model files
    switch(line_num)
        case 1
            model_x = 'models/model_l1px.h5';
            model_y = 'models/model_l1py.h5';
            model_z = 'models/model_l1pz.h5';
            model_xd = 'models/model_l1vx.h5';
            model_yd = 'models/model_l1vy.h5';
            model_zd = 'models/model_l1vz.h5';
        case 2
            model_x = 'models/model_l2px.h5';
            model_y = 'models/model_l2py.h5';
            model_z = 'models/model_l2pz.h5';
            model_xd = 'models/model_l2vx.h5';
            model_yd = 'models/model_l2vy.h5';
            model_zd = 'models/model_l2vz.h5';
        case 3
            model_x = 'models/model_l3px.h5';
            model_y = 'models/model_l3py.h5';
            model_z = 'models/model_l3pz.h5';
            model_xd = 'models/model_l3vx.h5';
            model_yd = 'models/model_l3vy.h5';
            model_zd = 'models/model_l3vz.h5';
        otherwise
            error('Invalid line number.');
    end
    
    % call surrogate model to predict positions and velocities
    x_py = py.predict_motions.predict_motions(model_x, inputs);
    y_py = py.predict_motions.predict_motions(model_y, inputs);
    z_py = py.predict_motions.predict_motions(model_z, inputs);
    xd_py = py.predict_motions.predict_motions(model_xd, inputs);
    yd_py = py.predict_motions.predict_motions(model_yd, inputs);
    zd_py = py.predict_motions.predict_motions(model_zd, inputs);

    % convert Python outputs to MATLAB data types
    x = double(x_py);
    y = double(y_py);
    z = double(z_py);
    xd = double(xd_py);
    yd = double(yd_py);
    zd = double(zd_py);

    
    
end

== matlab function HybridControllerP2C2ahm/Laboratory/MATLAB Function3 ==
  data: fx input; x output; fy input; fz input; elev input; line_num input; y output; z output; xd output; yd output; zd output
function [x, y, z, xd, yd, zd]  = SurrogateModel(fx, fy, fz, elev, line_num)
    
    % preallocate outputs
    x = double(0);
    y = double(0);
    z = double(0);
    xd = double(0);
    yd = double(0);
    zd = double(0);

    % declare python functions and inputs
    coder.extrinsic('py.list')
    coder.extrinsic('py.predict_motions.predict_motions');
    inputs = py.list({fx, fy, fz, elev});

    % set surrogate model files
    switch(line_num)
        case 1
            model_x = 'models/model_l1px.h5';
            model_y = 'models/model_l1py.h5';
            model_z = 'models/model_l1pz.h5';
            model_xd = 'models/model_l1vx.h5';
            model_yd = 'models/model_l1vy.h5';
            model_zd = 'models/model_l1vz.h5';
        case 2
            model_x = 'models/model_l2px.h5';
            model_y = 'models/model_l2py.h5';
            model_z = 'models/model_l2pz.h5';
            model_xd = 'models/model_l2vx.h5';
            model_yd = 'models/model_l2vy.h5';
            model_zd = 'models/model_l2vz.h5';
        case 3
            model_x = 'models/model_l3px.h5';
            model_y = 'models/model_l3py.h5';
            model_z = 'models/model_l3pz.h5';
            model_xd = 'models/model_l3vx.h5';
            model_yd = 'models/model_l3vy.h5';
            model_zd = 'models/model_l3vz.h5';
        otherwise
            error('Invalid line number.');
    end
    
    % call surrogate model to predict positions and velocities
    x_py = py.predict_motions.predict_motions(model_x, inputs);
    y_py = py.predict_motions.predict_motions(model_y, inputs);
    z_py = py.predict_motions.predict_motions(model_z, inputs);
    xd_py = py.predict_motions.predict_motions(model_xd, inputs);
    yd_py = py.predict_motions.predict_motions(model_yd, inputs);
    zd_py = py.predict_motions.predict_motions(model_zd, inputs);

    % convert Python outputs to MATLAB data types
    x = double(x_py);
    y = double(y_py);
    z = double(z_py);
    xd = double(xd_py);
    yd = double(yd_py);
    zd = double(zd_py);

end

== stateflow chart HybridControllerP2C2ahm/simPC HC/Predictor-Corrector ==
  state HybridController [parallel]
    settings: executionOrder=1
    state Initialize
      en:
      state = -1;
      i = 0; iSD = 0; diSD = 1;
      initData(nDOF,dtCon,dtSim,dtInt);
      state GetSetpoint
        en:
        setData(targSig);
        setSig(comSig,targSig);
        zeroSig(comSigDot);
        zeroSig(comSigDotDot);
        du:
        i = 0;
      (default) -> GetSetpoint
      GetSetpoint -> GetSetpoint : [after(dtCon,sec)]
          | {i=N;}
    state Correct
      en:
      state = 0;
      setCurSig(comSig,i/N);
      setNewSig(targSig);
      en, du:
      di = min(max(diSD+1/(0.1*N)*(i-iSD),0.001),1.0);
      i = min(i+di,N);
      correctD2(comSig,i/N);
      correctV2(comSigDot,i/N);
      correctA2(comSigDotDot,i/N);
    state Predict
      en:
      state = 1;
      setCurSig(comSig,1.0);
      i = 1; iSD = 0; diSD = 1;
      du:
      i++;
      en, du:
      predictD2(comSig,i/N);
      predictV2(comSigDot,i/N);
      predictA2(comSigDotDot,i/N);
    state AutoSlowDown
      en:
      state = 2;
      en, du:
      diSD = 9-i/(0.1*N); i += diSD; iSD = i;
      predictD2(comSig,i/N);
      predictV2(comSigDot,i/N);
      predictA2(comSigDotDot,i/N);
    Correct -> Predict [order 1] : [flag==0 && i==N]
    (default) -> Initialize
    Initialize -> Correct : [flag==1]
        | {i=0;}
    Predict -> Correct [order 2] : [flag==1]
    Predict -> AutoSlowDown [order 1] : [flag==0 && i>=0.8*N]
    AutoSlowDown -> Correct : [flag==1]
    Correct -> Correct [order 2] : [flag==1]
        | {i=0; iSD=0; diSD=1;}
  data: flag input int32; targSig input double size=nDOF+1; comSig output double size=nDOF+1; comSigDot output double size=nDOF+1; comSigDotDot output double size=nDOF+1; state output int32; i output double; N parameter int32; nDOF parameter int32; di local double; diSD local double; iSD local double; dtCon parameter double; dtSim parameter double; dtInt parameter double
